simulink model "task4_simulink"  (R2026a)
settings: Solver=VariableStepAuto  StopTime=20
settings Model: Creator=DELL  LastModifiedBy=DELL

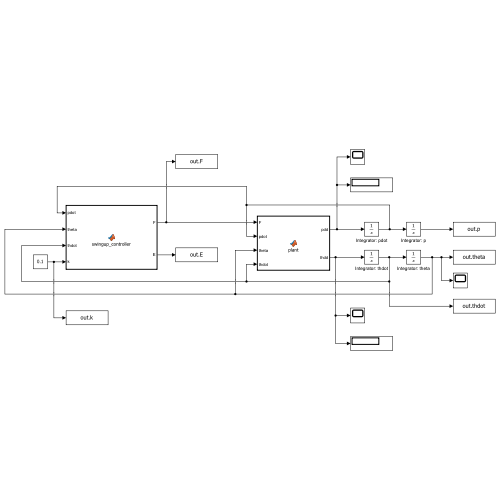
[thumbnail: Simulink's stored preview of the top-level diagram]
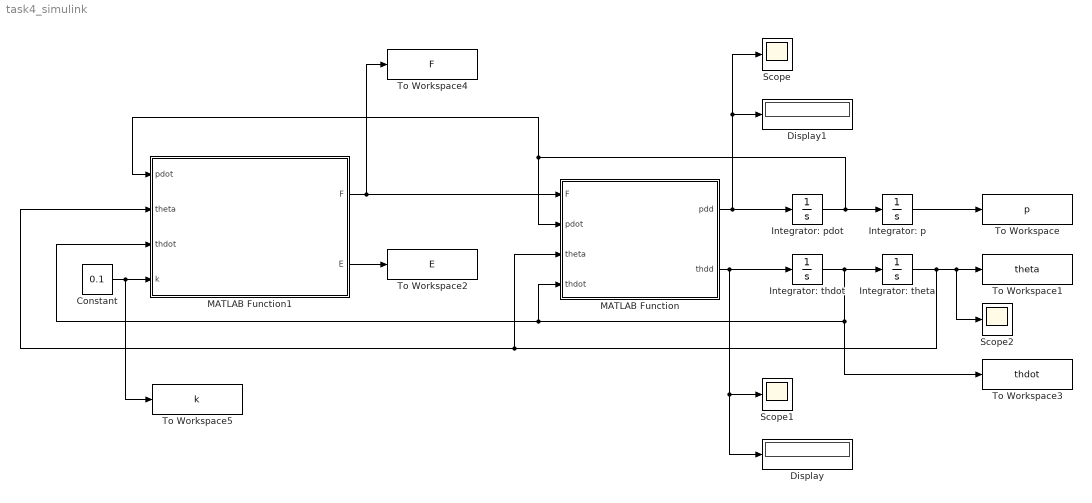
== system task4_simulink ==
  Constant : Constant  Value=0.1
  Display : Display
  Display1 : Display
  Integrator: p : Integrator
  Integrator: pdot : Integrator
  Integrator: thdot : Integrator
  Integrator: theta : Integrator  InitialCondition=pi-0.01
  MATLAB Function : MATLAB Function  TreatAsAtomicUnit=on
  MATLAB Function1 : MATLAB Function  TreatAsAtomicUnit=on
  Scope : Scope
      settings: ActiveDisplayYMinimum=-0.39641230245518316  ActiveDisplayYMaximum=0.44251737136425118
  Scope1 : Scope
      settings: ActiveDisplayYMinimum=-17.991162422784569  ActiveDisplayYMaximum=13.047383471679943
  Scope2 : Scope
      settings: ActiveDisplayYMinimum=-2.5099219897950631  ActiveDisplayYMaximum=10.897800353926344  DataLoggingVariableName=ScopeData2
  To Workspace : ToWorkspace  VariableName=p  SaveFormat=Timeseries  SampleTime=0.01
  To Workspace1 : ToWorkspace  VariableName=theta  SaveFormat=Timeseries  SampleTime=0.01
  To Workspace2 : ToWorkspace  VariableName=E  SaveFormat=Timeseries  SampleTime=0.01
  To Workspace3 : ToWorkspace  VariableName=thdot  SaveFormat=Timeseries  SampleTime=0.01
  To Workspace4 : ToWorkspace  VariableName=F  SaveFormat=Timeseries  SampleTime=0.01
  To Workspace5 : ToWorkspace  VariableName=k  SaveFormat=Timeseries  SampleTime=0.01
  wires:
  MATLAB Function/1(pdd) -> Display1/1, Scope/1, Integrator: pdot/1
  MATLAB Function/2(thdd) -> Display/1, Scope1/1, Integrator: thdot/1
  Integrator: pdot/1 -> MATLAB Function/2(pdot), MATLAB Function1/1(pdot), Integrator: p/1
  Integrator: thdot/1 -> MATLAB Function/4(thdot), MATLAB Function1/3(thdot), To Workspace3/1, Integrator: theta/1
  Integrator: theta/1 -> Scope2/1, To Workspace1/1, MATLAB Function/3(theta), MATLAB Function1/2(theta)
  Integrator: p/1 -> To Workspace/1
  MATLAB Function1/1(F) -> To Workspace4/1, MATLAB Function/1(F)
  MATLAB Function1/2(E) -> To Workspace2/1
  Constant/1 -> To Workspace5/1, MATLAB Function1/4(k)

== matlab function task4_simulink/MATLAB Function1 ==
  data: pdot input; F output; E output; theta input; thdot input; k input
function [F, E] = swingup_controller(pdot, theta, thdot, k)

M = 5;
m = 1;
l = 0.5;
c = 0.2;
g = 9.8;
Ed = 0;

E = 0.5*m*l^2*thdot^2 + m*g*l*(cos(theta)-1);
pdd_des = -k*(E-Ed)*thdot*cos(theta);
D = M+m-m*cos(theta)^2;
F = D*pdd_des + c*pdot - m*g*sin(theta)*cos(theta) + m*l*sin(theta)*thdot^2;

end

== matlab function task4_simulink/MATLAB Function ==
  data: F input; pdd output; pdot input; theta input; thdot input; thdd output
function [pdd, thdd] = plant(F, pdot, theta, thdot)

M = 5;
m = 1;
l = 0.5;
c = 0.2;
g = 9.8;

pdd = ( ...
    F ...
    - c*pdot ...
    + m*g*sin(theta)*cos(theta) ...
    - m*l*sin(theta)*thdot^2 ...
    ) / (M+m-m*cos(theta)^2);

thdd = ( ...
    cos(theta)*pdd ...
    + g*sin(theta) ...
    ) / l;

end
